simulink model "sf_superstep"  (R2025b)
settings: Solver=FixedStepDiscrete  StartTime=0.0  StopTime=10.0  FixedStep=1  RelTol=1e-3  EnableMultiTasking=on
settings Model: ExtModeAutoUpdateStatusClock=off  Creator=The MathWorks, Inc.  LastModifiedBy=The MathWorks, Inc.
settings SolverCC: AlgebraicLoopSolver=TrustRegion  InsertRTBMode=Auto
settings DataIOCC: LimitDataPoints=on  SaveFormat=Array  ReturnWorkspaceOutputs=off
settings OptimizationCC: ReuseModelBlockBuffer=off  ExpressionDepthLimit=2147483647.0  InitFltsAndDblsToZero=on  LifeSpan=inf
settings DebuggingCC: UnderspecifiedInitializationDetection=Classic  MergeDetectMultiDrivingBlocksExec=none  FcnCallInpInsideContextMsg=warning  UnconnectedInputMsg=warning  UnconnectedOutputMsg=warning  UnconnectedLineMsg=warning  StateNameClashWarn=warning  SFUnexpectedBacktrackingDiag=warning  SFNoUnconditionalDefaultTransitionDiag=warning  SFExecutionAtInitializationDiag=none  ArithmeticOperatorsInVariantConditions=warning
settings HardwareCC: ProdBitPerPointer=32.0  ProdBitPerSizeT=32.0  ProdBitPerPtrDiffT=32.0  ProdLargestAtomicFloat=None  ProdIntDivRoundTo=Undefined  ProdEndianess=Unspecified  ProdWordSize=32.0  ProdHWDeviceType=32-bit Generic
settings ModelReferenceCC: EnableRefExpFcnMdlSchedulingChecks=on  PropagateSignalLabelsOutOfModel=off
settings SFSimCC: SimUseLocalCustomCode=off  SimParseCustomCode=off  CustomCodeUndefinedFunction=UseInterfaceOnly
settings RTWCC: RTWUseLocalCustomCode=off  GPUComputeCapability=3.5  DLArmComputeVersion=19.05
settings CodeAppCC: StateflowObjectComments=on
settings GRTTargetCC: TargetLangStandard=C89/C90 (ANSI)  CombineOutputUpdateFcns=off  GRTInterface=on
settings ConfigComp: CovMetricSettings=dw  CovSaveCumulativeToWorkspaceVar=on  CovSaveSingleToWorkspaceVar=on  CovExternalEMLEnable=off  CovSFcnEnable=off

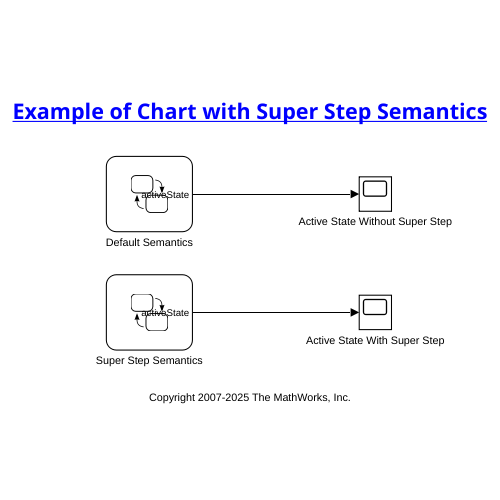
[thumbnail: Simulink's stored preview of the top-level diagram]
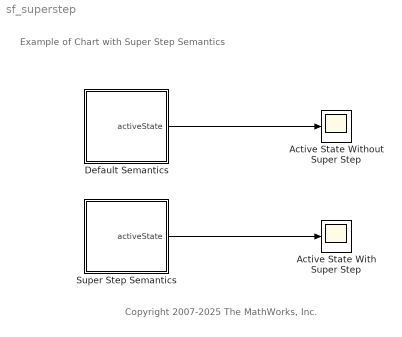
== system sf_superstep ==
  note: Copyright 2007-2025 The MathWorks, Inc.
  note: Example of Chart with Super Step Semantics
  Active State With Super Step : Scope
      settings: ActiveDisplayYMinimum=0.75  ActiveDisplayYMaximum=3.25
  Active State Without Super Step : Scope
      settings: ActiveDisplayYMinimum=0.75  ActiveDisplayYMaximum=3.25
  Default Semantics : Stateflow chart  TreatAsAtomicUnit=on
  Super Step Semantics : Stateflow chart  TreatAsAtomicUnit=on
  wires:
  Default Semantics/1(activeState) -> Active State Without Super Step/1
  Super Step Semantics/1(activeState) -> Active State With Super Step/1

== stateflow chart sf_superstep/Default Semantics ==
  state A
  state B
  state C
  (default) -> A
  B -> C
  A -> B
  data: activeState output Enum: chartType

== stateflow chart sf_superstep/Super Step Semantics ==
  settings: enableNonTerminalStates=1
  state A
  state B
  state C
  (default) -> A
  B -> C
  A -> B
  data: activeState output Enum: chartType
